simulink model "conjunction_sim"  (R2024b)
settings: Solver=ode113  StartTime=0  StopTime=T_lead  RelTol=ode_reltol  AbsTol=ode_abstol
undefined symbols (not defined in the file): burn_sign, burns, mu_earth, r1_0, r2_0, u_draw, v1_0, v2_0, x_rule_flat
settings Model: Creator=PC  LastModifiedBy=PC
settings DataIOCC: SaveOutput=off  SignalLogging=off

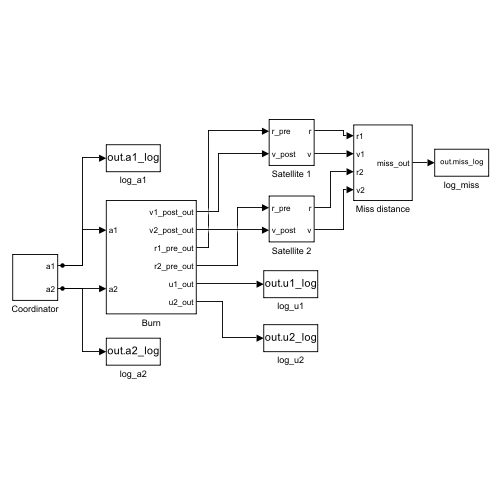
[thumbnail: Simulink's stored preview of the top-level diagram]
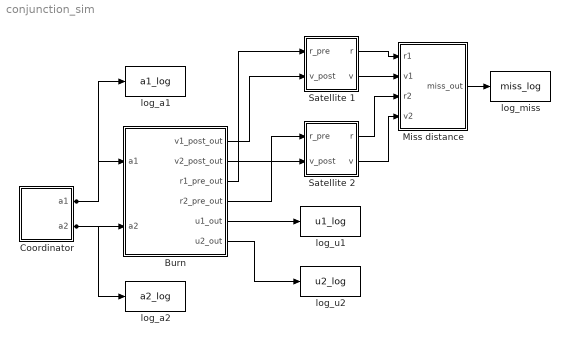
== system conjunction_sim ==
  Burn : Subsystem
  Coordinator : Subsystem
  Miss distance : Subsystem
  Satellite 1 : Subsystem
  Satellite 2 : Subsystem
  log_a1 : ToWorkspace  VariableName=a1_log  SampleTime=-1
  log_a2 : ToWorkspace  VariableName=a2_log  SampleTime=-1
  log_miss : ToWorkspace  VariableName=miss_log  SampleTime=-1
  log_u1 : ToWorkspace  VariableName=u1_log  SampleTime=-1
  log_u2 : ToWorkspace  VariableName=u2_log  SampleTime=-1
  wires:
  Coordinator/2(a2) -> Burn/2(a2), log_a2/1
  Coordinator/1(a1) -> Burn/1(a1), log_a1/1
  Burn/1(v1_post_out) -> Satellite 1/2(v_post)
  Burn/5(u1_out) -> log_u1/1
  Burn/3(r1_pre_out) -> Satellite 1/1(r_pre)
  Burn/4(r2_pre_out) -> Satellite 2/1(r_pre)
  Burn/2(v2_post_out) -> Satellite 2/2(v_post)
  Burn/6(u2_out) -> log_u2/1
  Satellite 1/1(r) -> Miss distance/1(r1)
  Satellite 1/2(v) -> Miss distance/2(v1)
  Satellite 2/1(r) -> Miss distance/3(r2)
  Satellite 2/2(v) -> Miss distance/4(v2)
  Miss distance/1(miss_out) -> log_miss/1

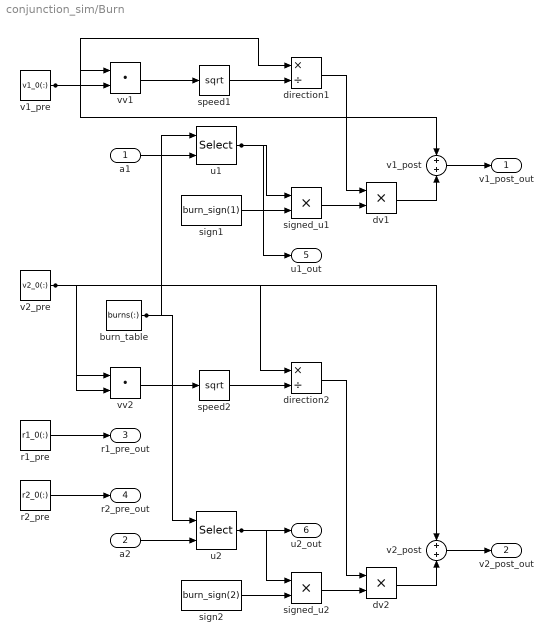
== system conjunction_sim/Burn ==
  a1 : Inport
  a2 : Inport  Port=2
  burn_table : Constant  Value=burns(:)
  direction1 : Product  Inputs=*/
  direction2 : Product  Inputs=*/
  dv1 : Product  Inputs=**
  dv2 : Product  Inputs=**
  r1_pre : Constant  Value=r1_0(:)
  r2_pre : Constant  Value=r2_0(:)
  sign1 : Constant  Value=burn_sign(1)
  sign2 : Constant  Value=burn_sign(2)
  signed_u1 : Product  Inputs=**
  signed_u2 : Product  Inputs=**
  speed1 : Sqrt
  speed2 : Sqrt
  u1 : Selector  IndexOptions=Index vector (port)  Indices=[1 3]  OutputSizes=1
  u2 : Selector  IndexOptions=Index vector (port)  Indices=[1 3]  OutputSizes=1
  v1_post : Sum
  v1_pre : Constant  Value=v1_0(:)
  v2_post : Sum
  v2_pre : Constant  Value=v2_0(:)
  vv1 : DotProduct  OutDataTypeStr=Inherit: Inherit via internal rule
  vv2 : DotProduct  OutDataTypeStr=Inherit: Inherit via internal rule
  v1_post_out : Outport
  v2_post_out : Outport  Port=2
  r1_pre_out : Outport  Port=3
  r2_pre_out : Outport  Port=4
  u1_out : Outport  Port=5
  u2_out : Outport  Port=6
  wires:
  r1_pre/1 -> r1_pre_out/1
  burn_table/1 -> u1/1, u2/1
  v1_pre/1 -> direction1/1, vv1/2, vv1/1, v1_post/1
  a1/1 -> u1/2
  r2_pre/1 -> r2_pre_out/1
  v2_pre/1 -> direction2/1, v2_post/1, vv2/1, vv2/2
  vv1/1 -> speed1/1
  vv2/1 -> speed2/1
  a2/1 -> u2/2
  dv1/1 -> v1_post/2
  direction1/1 -> dv1/1
  speed1/1 -> direction1/2
  sign2/1 -> signed_u2/2
  u1/1 -> signed_u1/1, u1_out/1
  signed_u1/1 -> dv1/2
  sign1/1 -> signed_u1/2
  dv2/1 -> v2_post/2
  speed2/1 -> direction2/2
  u2/1 -> signed_u2/1, u2_out/1
  v2_post/1 -> v2_post_out/1
  direction2/1 -> dv2/1
  signed_u2/1 -> dv2/2
  v1_post/1 -> v1_post_out/1

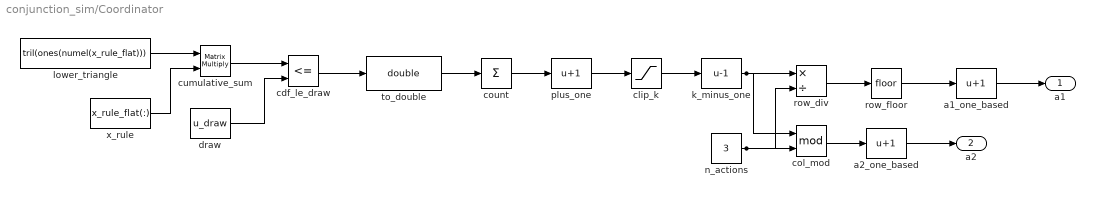
== system conjunction_sim/Coordinator ==
  a1_one_based : Bias  Bias=1  SaturateOnIntegerOverflow=off
  a2_one_based : Bias  Bias=1  SaturateOnIntegerOverflow=off
  cdf_le_draw : RelationalOperator  Operator=<=  OutDataTypeStr=boolean  RndMeth=Simplest  InputSameDT=off
  clip_k : Saturate  UpperLimit=numel(x_rule_flat)  LowerLimit=1
  col_mod : Math  Operator=mod
  count : Sum  Inputs=+
  cumulative_sum : Product  Multiplication=Matrix(*)
  draw : Constant  Value=u_draw
  k_minus_one : Bias  Bias=-1  SaturateOnIntegerOverflow=off
  lower_triangle : Constant  Value=tril(ones(numel(x_rule_flat)))
  n_actions : Constant  Value=3
  plus_one : Bias  Bias=1  SaturateOnIntegerOverflow=off
  row_div : Product  Inputs=*/
  row_floor : Rounding
  to_double : DataTypeConversion  OutDataTypeStr=double  SaturateOnIntegerOverflow=off  RndMeth=Floor
  x_rule : Constant  Value=x_rule_flat(:)
  a1 : Outport
  a2 : Outport  Port=2
  wires:
  lower_triangle/1 -> cumulative_sum/1
  x_rule/1 -> cumulative_sum/2
  draw/1 -> cdf_le_draw/2
  cumulative_sum/1 -> cdf_le_draw/1
  row_div/1 -> row_floor/1
  count/1 -> plus_one/1
  to_double/1 -> count/1
  cdf_le_draw/1 -> to_double/1
  n_actions/1 -> row_div/2, col_mod/2
  plus_one/1 -> clip_k/1
  clip_k/1 -> k_minus_one/1
  k_minus_one/1 -> row_div/1, col_mod/1
  col_mod/1 -> a2_one_based/1
  row_floor/1 -> a1_one_based/1
  a2_one_based/1 -> a2/1
  a1_one_based/1 -> a1/1

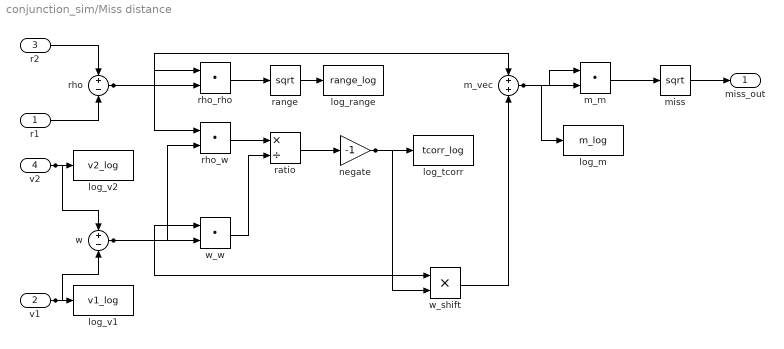
== system conjunction_sim/Miss distance ==
  r1 : Inport
  v1 : Inport  Port=2
  r2 : Inport  Port=3
  v2 : Inport  Port=4
  log_m : ToWorkspace  VariableName=m_log  SampleTime=-1
  log_range : ToWorkspace  VariableName=range_log  SampleTime=-1
  log_tcorr : ToWorkspace  VariableName=tcorr_log  SampleTime=-1
  log_v1 : ToWorkspace  VariableName=v1_log  SampleTime=-1
  log_v2 : ToWorkspace  VariableName=v2_log  SampleTime=-1
  m_m : DotProduct  OutDataTypeStr=Inherit: Inherit via internal rule
  m_vec : Sum
  miss : Sqrt
  negate : Gain  Gain=-1
  range : Sqrt
  ratio : Product  Inputs=*/
  rho : Sum  Inputs=+-
  rho_rho : DotProduct  OutDataTypeStr=Inherit: Inherit via internal rule
  rho_w : DotProduct  OutDataTypeStr=Inherit: Inherit via internal rule
  w : Sum  Inputs=+-
  w_shift : Product  Inputs=**
  w_w : DotProduct  OutDataTypeStr=Inherit: Inherit via internal rule
  miss_out : Outport
  wires:
  v1/1 -> w/2, log_v1/1
  r1/1 -> rho/2
  r2/1 -> rho/1
  rho/1 -> rho_w/1, rho_rho/1, rho_rho/2, m_vec/1
  v2/1 -> w/1, log_v2/1
  rho_w/1 -> ratio/1
  rho_rho/1 -> range/1
  w/1 -> w_w/1, w_w/2, rho_w/2, w_shift/1
  range/1 -> log_range/1
  w_w/1 -> ratio/2
  ratio/1 -> negate/1
  m_vec/1 -> m_m/1, m_m/2, log_m/1
  negate/1 -> w_shift/2, log_tcorr/1
  m_m/1 -> miss/1
  w_shift/1 -> m_vec/2
  miss/1 -> miss_out/1

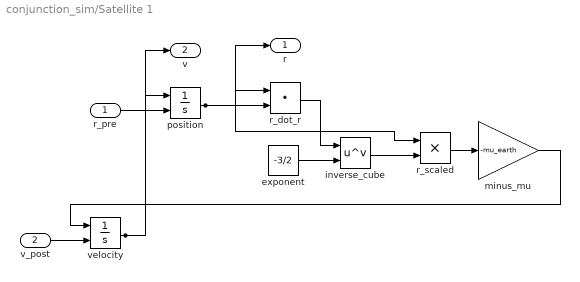
== system conjunction_sim/Satellite 1 ==
  r_pre : Inport
  v_post : Inport  Port=2
  exponent : Constant  Value=-3/2
  inverse_cube : Math  Operator=pow
  minus_mu : Gain  Gain=-mu_earth
  position : Integrator  InitialConditionSource=external
  r_dot_r : DotProduct  OutDataTypeStr=Inherit: Inherit via internal rule
  r_scaled : Product  Inputs=**
  velocity : Integrator  InitialConditionSource=external
  r : Outport
  v : Outport  Port=2
  wires:
  r_pre/1 -> position/2
  v_post/1 -> velocity/2
  exponent/1 -> inverse_cube/2
  r_dot_r/1 -> inverse_cube/1
  position/1 -> r_scaled/1, r_dot_r/1, r/1, r_dot_r/2
  velocity/1 -> position/1, v/1
  r_scaled/1 -> minus_mu/1
  inverse_cube/1 -> r_scaled/2
  minus_mu/1 -> velocity/1

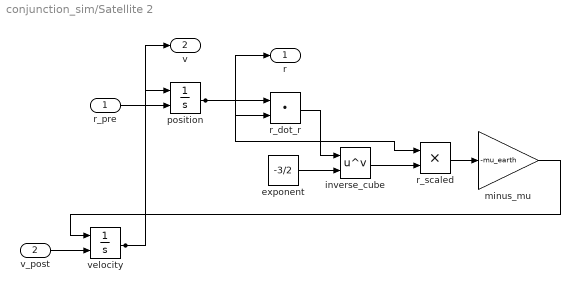
== system conjunction_sim/Satellite 2 ==
  r_pre : Inport
  v_post : Inport  Port=2
  exponent : Constant  Value=-3/2
  inverse_cube : Math  Operator=pow
  minus_mu : Gain  Gain=-mu_earth
  position : Integrator  InitialConditionSource=external
  r_dot_r : DotProduct  OutDataTypeStr=Inherit: Inherit via internal rule
  r_scaled : Product  Inputs=**
  velocity : Integrator  InitialConditionSource=external
  r : Outport
  v : Outport  Port=2
  wires:
  exponent/1 -> inverse_cube/2
  r_scaled/1 -> minus_mu/1
  inverse_cube/1 -> r_scaled/2
  r_dot_r/1 -> inverse_cube/1
  v_post/1 -> velocity/2
  position/1 -> r_scaled/1, r_dot_r/2, r_dot_r/1, r/1
  r_pre/1 -> position/2
  velocity/1 -> position/1, v/1
  minus_mu/1 -> velocity/1
